simulink library "RollHeave_Decoupled"  (R2025a)
settings: Solver=VariableStepAuto  StartTime=0.0  StopTime=10.0  RelTol=1e-3
undefined symbols (not defined in the file): Linkage, Visual, X, Y, Z
libraries: Suspension_Utilities x12, sm_lib x8, nesl_utility x4, Linkage_Shock x2
Description:
  | Component of Simscape Vehicle Templates Library
  | 
  | Copyright 2018-2026 The MathWorks, Inc.
settings Model: Creator=smiller  LastModifiedBy=smiller
settings SolverCC: AlgebraicLoopSolver=TrustRegion
settings DataIOCC: ReturnWorkspaceOutputs=off
settings OptimizationCC: ReuseModelBlockBuffer=off
settings DebuggingCC: UnconnectedInputMsg=warning  UnconnectedOutputMsg=warning  UnconnectedLineMsg=warning  ArithmeticOperatorsInVariantConditions=warning
settings ModelReferenceCC: EnableRefExpFcnMdlSchedulingChecks=on
settings SFSimCC: CustomCodeUndefinedFunction=UseInterfaceOnly
settings RTWCC: GPUComputeCapability=3.5

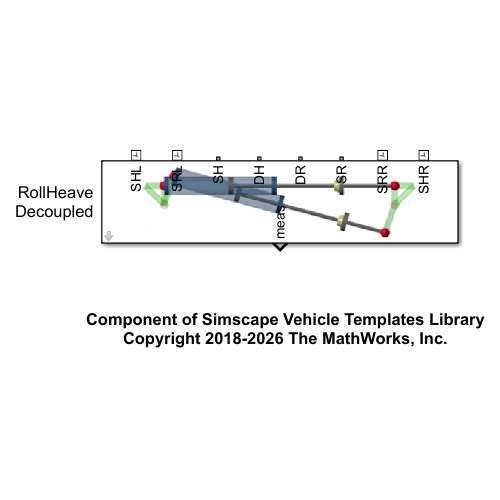
[thumbnail: Simulink's stored preview of the top-level diagram]
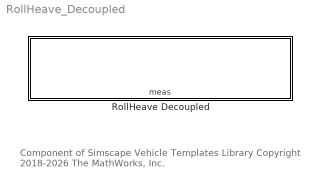
== system RollHeave_Decoupled ==
  note: Component of Simscape Vehicle Templates Library
      | Copyright 2018-2026 The MathWorks, Inc.
  RollHeave Decoupled : Subsystem  VariantControl=Variant1  mask(Roll and Heave Spring Dampers){hp_pushrod=Linkage.Pushrod.sBellcrank.Value, hp_bcr_pivot=Linkage.Bellcrank.sPivot.Value, hp_bcr_shock_heaveL=Linkage.Shock.Heave.sLeft.Value, hp_bcr_shock_heaveR=Linkage.Shock.Heave.sRight.Value, hp_bcr_shock_rollL=Linkage.Shock.Roll.sLeft.Value, hp_bcr_shock_rollR=Linkage.Shock.Roll.sRight.Value, shock_pist_mass_heave=Linkage.Shock.Heave.mPiston.Value, shock_pist_mass_roll=Linkage.Shock.Roll.mPiston.Value, shock_cyl_mass_heave=Linkage.Shock.Heave.mCylinder.Value, shock_cyl_mass_roll=Linkage.Shock.Roll.mCylinder.Value, up_lim_bumpstop_heave=Linkage.Endstop.Heave.xMax.Value, up_lim_bumpstop_roll=Linkage.Endstop.Roll.xMax.Value, low_lim_bumpstop_heave=Linkage.Endstop.Heave.xMin.Value, low_lim_bumpstop_roll=Linkage.Endstop.Roll.xMin.Value, clr_conn_shock=Visual.hp.clr, opc_conn_shock=Visual.hp.opc, size_conn_shock=Visual.hp.rad, clr_shock_cyl=Visual.Shock.cyl.clr, opc_shock_cyl=Visual.part.opc, radius_shock_cyl=Visual.Shock.cyl.rad, clr_shock_piston=Visual.Shock.piston.clr, opc_shock_piston=Visual.part.opc, clr_shock_bumpstop=Visual.Shock.bumpstop.clr, opc_shock_bumpstop=Visual.part.opc, deadvol_len_shock_cyl=Visual.Shock.dead_length, piston_len_shock=Visual.Shock.piston.len, cyl_cap_len_shock=Visual.Shock.cap.len, bumpstop_len_shock=Visual.Shock.bumpstop.len}
      mask prompts: hp_pushrod "HP Pushrod Inner  [xyz] (m)"; hp_bcr_pivot "HP Bellcrank Pivot [xyz] (m)"; deadvol_len_shock_cyl "Dead Volume Height (m)"; piston_len_shock "Piston Length (m)"; cyl_cap_len_shock "Cylinder Cap Length (m)"; bumpstop_len_shock "Bumpstop Length (m)"
      mask help: Models springs and dampers in a suspension design that decouples stiffness and damping for body roll and heave.
      mask init:
      | % Code to mirror hardpoint about vehicle xz plane
      | % and the plane defined by the bellcrank pivot axis
      | % and the y axis of the vehicle
      | % Code not used so that points can be specified independently
      | % Left here as a reference.
      | %{
      |  
      | a1 = atan2(hp_pushrod(1)-hp_bcr_pivot(1)   ,hp_pushrod(3)-hp_bcr_pivot(3));
      | a2 = atan2(hp_bcr_shock_roll(1)-hp_bcr_pivot(1),hp_bcr_shock_roll(3)-hp_bcr_pivot(3));
      | d_roll2piv = norm(hp_bcr_shock_roll([1 3])-hp_bcr_pivot([1 3]));
      | d_roll_mirror_axis = d_roll2piv*cos(a2-a1);
      | mirr_dx = d_roll_mirror_axis*sin(a1);
      | mirr_dz = d_roll_mirror_axis*cos(a1);
      | hp_bcr_shock_roll_r = ...
      |     [hp_bcr_shock_roll(1)-2*mirr_dx -hp_bcr_shock_roll(2) hp_bcr_shock_roll(3)-2*mirr_dz]
      | %}
      mask TypeOptions shock_pist_mass_heave: Shock Heave/shock_pist_mass
      mask TypeOptions shock_pist_mass_roll: Shock Roll/shock_pist_mass
      mask TypeOptions shock_cyl_mass_heave: Shock Heave/shock_cyl_mass
      mask TypeOptions shock_cyl_mass_roll: Shock Roll/shock_cyl_mass
      mask TypeOptions up_lim_bumpstop_heave: Shock Heave/up_lim_bumpstop
      mask TypeOptions up_lim_bumpstop_roll: Shock Roll/up_lim_bumpstop
      mask TypeOptions low_lim_bumpstop_heave: Shock Heave/low_lim_bumpstop
      mask TypeOptions low_lim_bumpstop_roll: Shock Roll/low_lim_bumpstop
      mask TypeOptions clr_conn_shock: Shock Heave/clr_conn_shock | Shock Roll/clr_conn_shock
      mask TypeOptions opc_conn_shock: Shock Heave/opc_conn_shock | Shock Roll/opc_conn_shock
      mask TypeOptions size_conn_shock: Shock Heave/size_conn_shock | Shock Roll/size_conn_shock
      mask TypeOptions clr_shock_cyl: Shock Heave/clr_shock_cyl | Shock Roll/clr_shock_cyl
      mask TypeOptions opc_shock_cyl: Shock Heave/opc_shock_cyl | Shock Roll/opc_shock_cyl
      mask TypeOptions radius_shock_cyl: Shock Heave/radius_shock_cyl | Shock Roll/radius_shock_cyl
      mask TypeOptions clr_shock_piston: Shock Heave/clr_shock_piston | Shock Roll/clr_shock_piston
      mask TypeOptions opc_shock_piston: Shock Heave/opc_shock_piston | Shock Roll/opc_shock_piston
      mask TypeOptions clr_shock_bumpstop: Shock Heave/clr_shock_bumpstop | Shock Roll/clr_shock_bumpstop
      mask TypeOptions opc_shock_bumpstop: Shock Heave/opc_shock_bumpstop | Shock Roll/opc_shock_bumpstop
      mask TypeOptions deadvol_len_shock_cyl: Shock Heave/deadvol_len_shock_cyl | Shock Roll/deadvol_len_shock_cyl
      mask TypeOptions piston_len_shock: Shock Heave/piston_len_shock | Shock Roll/piston_len_shock
      mask TypeOptions cyl_cap_len_shock: Shock Heave/cyl_cap_len_shock | Shock Roll/cyl_cap_len_shock
      mask TypeOptions bumpstop_len_shock: Shock Heave/bumpstop_len_shock | Shock Roll/bumpstop_len_shock
      mask DialogControl cont_hp Prompt: Hardpoints
      mask DialogControl text_hp_left Prompt: Left
      mask DialogControl text_hp_right Prompt: Right
      mask DialogControl text_hp_heave Prompt: Heave [xyz] (m)
      mask DialogControl text_hp_roll Prompt: Roll [xyz] (m)
      mask DialogControl cont_shock Prompt: Shock
      mask DialogControl text_shock_parts_blank Prompt: Parts
      mask DialogControl text_shock_heave Prompt: Heave
      mask DialogControl text_shock_roll Prompt: Roll
      mask DialogControl text_shock_pistm Prompt: Piston Mass (kg)
      mask DialogControl text_shock_cylm Prompt: Cylinder Mass (kg)
      mask DialogControl text_shock_bumpstop_par Prompt: Bumpstop
      mask DialogControl text_bump_ul Prompt: Upper Limit (m)
      mask DialogControl text_bump_low Prompt: Lower Limit (m)
      mask DialogControl cont_vis_shock Prompt: Visualization
      mask DialogControl text_clr_shock Prompt: Color  [RGB]
      mask DialogControl text_opc_shock Prompt: Opac. (0-1)
      mask DialogControl text_size_shock Prompt: Size (m)
      mask DialogControl text_conn_shock Prompt: Connections
      mask DialogControl text_shock_shock Prompt: Cylinder
      mask DialogControl text_shock_piston Prompt: Piston
      mask DialogControl text_piston_radius Prompt: <cylinder radius>
      mask DialogControl text_shock_bumpstop Prompt: Bumpstop
      mask DialogControl text_bumpstop_radius Prompt: <cylinder radius>
      mask Display: image('sm_car_vehicle_linkage_rollHeaveDecouple_IMAGE.png');

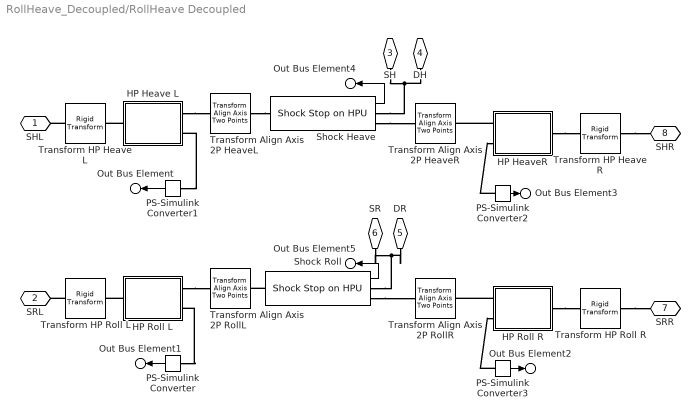
== system RollHeave_Decoupled/RollHeave Decoupled ==
  HP Heave L : Subsystem  mask(Revolute Joint 3 Points){popup_leftRight=Left, hp_bcr_pivot=hp_bcr_pivot, hp_pushrod_in=hp_pushrod, hp_bcr_shock=hp_bcr_shock_heaveL}
      mask prompts: popup_leftRight "Left/Right"; hp_bcr_pivot "HP Bellcrank Pivot [xyz] (m)"; hp_pushrod_in "HP Pushrod Inner [xyz] (m)"; hp_bcr_shock "HP Bellcrank Shock Heave [xyz] (m)"
      mask help: Revolute Joint with degree of freedom normal to 3 hardpoints.
      mask init:
      | % Set parameter for mirroring (+y or -y)
      | if(popup_leftRight == 1)
      |     rhs_susp = 1;    
      | elseif(popup_leftRight == 2)
      |     rhs_susp = -1;
      | end
      | 
      | rhs_hp = [1 rhs_susp 1];
      mask TypeOptions popup_leftRight: Left | Right
      mask Display: image('sm_car_variant_revolute.png')
  HP HeaveR : Subsystem  mask(Revolute Joint 3 Points){popup_leftRight=Right, hp_bcr_pivot=hp_bcr_pivot, hp_pushrod_in=hp_pushrod, hp_bcr_shock=hp_bcr_shock_heaveR}
      mask prompts: popup_leftRight "Left/Right"; hp_bcr_pivot "HP Bellcrank Pivot [xyz] (m)"; hp_pushrod_in "HP Pushrod Inner [xyz] (m)"; hp_bcr_shock "HP Bellcrank Shock Heave [xyz] (m)"
      mask help: Revolute Joint with degree of freedom normal to 3 hardpoints.
      mask init:
      | % Set parameter for mirroring (+y or -y)
      | if(popup_leftRight == 1)
      |     rhs_susp = 1;    
      | elseif(popup_leftRight == 2)
      |     rhs_susp = -1;
      | end
      | 
      | rhs_hp = [1 rhs_susp 1];
      mask TypeOptions popup_leftRight: Left | Right
      mask Display: image('sm_car_variant_revolute.png')
  HP Roll L : Subsystem  mask(Revolute Joint 3 Points){popup_leftRight=Left, hp_bcr_pivot=hp_bcr_pivot, hp_pushrod_in=hp_pushrod, hp_bcr_shock=hp_bcr_shock_heaveL}
      mask prompts: popup_leftRight "Left/Right"; hp_bcr_pivot "HP Bellcrank Pivot [xyz] (m)"; hp_pushrod_in "HP Pushrod Inner [xyz] (m)"; hp_bcr_shock "HP Bellcrank Shock Heave [xyz] (m)"
      mask help: Revolute Joint with degree of freedom normal to 3 hardpoints.
      mask init:
      | % Set parameter for mirroring (+y or -y)
      | if(popup_leftRight == 1)
      |     rhs_susp = 1;    
      | elseif(popup_leftRight == 2)
      |     rhs_susp = -1;
      | end
      | 
      | rhs_hp = [1 rhs_susp 1];
      mask TypeOptions popup_leftRight: Left | Right
      mask Display: image('sm_car_variant_revolute.png')
  HP Roll R : Subsystem  mask(Revolute Joint 3 Points){popup_leftRight=Right, hp_bcr_pivot=hp_bcr_pivot, hp_pushrod_in=hp_pushrod, hp_bcr_shock=hp_bcr_shock_heaveR}
      mask prompts: popup_leftRight "Left/Right"; hp_bcr_pivot "HP Bellcrank Pivot [xyz] (m)"; hp_pushrod_in "HP Pushrod Inner [xyz] (m)"; hp_bcr_shock "HP Bellcrank Shock Heave [xyz] (m)"
      mask help: Revolute Joint with degree of freedom normal to 3 hardpoints.
      mask init:
      | % Set parameter for mirroring (+y or -y)
      | if(popup_leftRight == 1)
      |     rhs_susp = 1;    
      | elseif(popup_leftRight == 2)
      |     rhs_susp = -1;
      | end
      | 
      | rhs_hp = [1 rhs_susp 1];
      mask TypeOptions popup_leftRight: Left | Right
      mask Display: image('sm_car_variant_revolute.png')
  PS-Simulink Converter{,1..3} (4 alike) : nesl_utility/PS-Simulink Converter  PhysicalDomain=network_engine_domain  SubClassName=ps_output  LeftPortType=input  RightPortType=output  PseudoPeriodic=off  Frequencies=[]  VectorFormat=1-D array  Unit=1  AffineConversion=off
  Shock Heave : Linkage_Shock/Shock Stop on HPU  shock_pist_mass=shock_pist_mass_heave  shock_cyl_mass=shock_cyl_mass_heave  hp_spr_top=hp_bcr_shock_heaveR  hp_spr_bot=hp_bcr_shock_heaveL  up_lim_bumpstop=up_lim_bumpstop_heave  low_lim_bumpstop=low_lim_bumpstop_heave  clr_conn_shock=clr_conn_shock  opc_conn_shock=opc_conn_shock  size_conn_shock=size_conn_shock  clr_shock_cyl=clr_shock_cyl  opc_shock_cyl=opc_shock_cyl  radius_shock_cyl=radius_shock_cyl  clr_shock_piston=clr_shock_piston  opc_shock_piston=opc_shock_piston  clr_shock_bumpstop=clr_shock_bumpstop  opc_shock_bumpstop=opc_shock_bumpstop  deadvol_len_shock_cyl=deadvol_len_shock_cyl  piston_len_shock=piston_len_shock  cyl_cap_len_shock=cyl_cap_len_shock  bumpstop_len_shock=bumpstop_len_shock
  Shock Roll : Linkage_Shock/Shock Stop on HPU  shock_pist_mass=shock_pist_mass_roll  shock_cyl_mass=shock_cyl_mass_roll  hp_spr_top=hp_bcr_shock_rollR  hp_spr_bot=hp_bcr_shock_rollL  up_lim_bumpstop=up_lim_bumpstop_roll  low_lim_bumpstop=low_lim_bumpstop_roll  clr_conn_shock=clr_conn_shock  opc_conn_shock=opc_conn_shock  size_conn_shock=size_conn_shock  clr_shock_cyl=clr_shock_cyl  opc_shock_cyl=opc_shock_cyl  radius_shock_cyl=radius_shock_cyl  clr_shock_piston=clr_shock_piston  opc_shock_piston=opc_shock_piston  clr_shock_bumpstop=clr_shock_bumpstop  opc_shock_bumpstop=opc_shock_bumpstop  deadvol_len_shock_cyl=deadvol_len_shock_cyl  piston_len_shock=piston_len_shock  cyl_cap_len_shock=cyl_cap_len_shock  bumpstop_len_shock=bumpstop_len_shock
  Transform Align Axis 2P HeaveL : Suspension_Utilities/Transform Align Axis Two Points  hp_b=hp_bcr_shock_heaveL  hp_t=hp_bcr_shock_heaveR  popup_f_axis=+Z
  Transform Align Axis 2P HeaveR : Suspension_Utilities/Transform Align Axis Two Points  hp_b=hp_bcr_shock_heaveR  hp_t=hp_bcr_shock_heaveL  popup_f_axis=-Z
  Transform Align Axis 2P RollL : Suspension_Utilities/Transform Align Axis Two Points  hp_b=hp_bcr_shock_rollL  hp_t=hp_bcr_shock_rollR  popup_f_axis=+Z
  Transform Align Axis 2P RollR : Suspension_Utilities/Transform Align Axis Two Points  hp_b=hp_bcr_shock_rollR  hp_t=hp_bcr_shock_rollL  popup_f_axis=-Z
  "Transform HP Heave L " : sm_lib/Frames and Transforms/Rigid Transform  RotationMethod=None  FollAlignAxisA=+X  BaseAlignAxisA=+Y  FollAlignAxisB=+Y  BaseAlignAxisB=+Z  RotationStandardAxis=+Z  RotationAngle=0.0  RotationAngleUnits=deg  RotationArbitraryAxis=[0 0 1]  RotationSequenceAxes=FollowerAxes  RotationSequence=XYX  RotationSequenceAngles=[0 0 0]  RotationSequenceAnglesUnits=deg  RotationMatrix=[1 0 0; 0 1 0; 0 0 1]  Quaternion=[1 0 0 0]  TranslationMethod=Cartesian  TranslationCartesianOffset=hp_bcr_shock_heaveL  TranslationCartesianOffsetUnits=m  TranslationStandardAxis=+Z  TranslationStandardOffset=0  TranslationStandardOffsetUnits=m  TranslationROffset=0  TranslationROffsetUnits=m  TranslationThetaOffset=0  TranslationThetaOffsetUnits=deg  TranslationZOffset=0  TranslationZOffsetUnits=m
  Transform HP Heave R : sm_lib/Frames and Transforms/Rigid Transform  RotationMethod=None  FollAlignAxisA=+X  BaseAlignAxisA=+Y  FollAlignAxisB=+Y  BaseAlignAxisB=+Z  RotationStandardAxis=+Z  RotationAngle=0.0  RotationAngleUnits=deg  RotationArbitraryAxis=[0 0 1]  RotationSequenceAxes=FollowerAxes  RotationSequence=XYX  RotationSequenceAngles=[0 0 0]  RotationSequenceAnglesUnits=deg  RotationMatrix=[1 0 0; 0 1 0; 0 0 1]  Quaternion=[1 0 0 0]  TranslationMethod=Cartesian  TranslationCartesianOffset=hp_bcr_shock_heaveR  TranslationCartesianOffsetUnits=m  TranslationStandardAxis=+Z  TranslationStandardOffset=0  TranslationStandardOffsetUnits=m  TranslationROffset=0  TranslationROffsetUnits=m  TranslationThetaOffset=0  TranslationThetaOffsetUnits=deg  TranslationZOffset=0  TranslationZOffsetUnits=m
  Transform HP Roll L : sm_lib/Frames and Transforms/Rigid Transform  RotationMethod=None  FollAlignAxisA=+X  BaseAlignAxisA=+Y  FollAlignAxisB=+Y  BaseAlignAxisB=+Z  RotationStandardAxis=+Z  RotationAngle=0.0  RotationAngleUnits=deg  RotationArbitraryAxis=[0 0 1]  RotationSequenceAxes=FollowerAxes  RotationSequence=XYX  RotationSequenceAngles=[0 0 0]  RotationSequenceAnglesUnits=deg  RotationMatrix=[1 0 0; 0 1 0; 0 0 1]  Quaternion=[1 0 0 0]  TranslationMethod=Cartesian  TranslationCartesianOffset=hp_bcr_shock_rollL  TranslationCartesianOffsetUnits=m  TranslationStandardAxis=+Z  TranslationStandardOffset=0  TranslationStandardOffsetUnits=m  TranslationROffset=0  TranslationROffsetUnits=m  TranslationThetaOffset=0  TranslationThetaOffsetUnits=deg  TranslationZOffset=0  TranslationZOffsetUnits=m
  Transform HP Roll R : sm_lib/Frames and Transforms/Rigid Transform  RotationMethod=None  FollAlignAxisA=+X  BaseAlignAxisA=+Y  FollAlignAxisB=+Y  BaseAlignAxisB=+Z  RotationStandardAxis=+Z  RotationAngle=0.0  RotationAngleUnits=deg  RotationArbitraryAxis=[0 0 1]  RotationSequenceAxes=FollowerAxes  RotationSequence=XYX  RotationSequenceAngles=[0 0 0]  RotationSequenceAnglesUnits=deg  RotationMatrix=[1 0 0; 0 1 0; 0 0 1]  Quaternion=[1 0 0 0]  TranslationMethod=Cartesian  TranslationCartesianOffset=hp_bcr_shock_rollR  TranslationCartesianOffsetUnits=m  TranslationStandardAxis=+Z  TranslationStandardOffset=0  TranslationStandardOffsetUnits=m  TranslationROffset=0  TranslationROffsetUnits=m  TranslationThetaOffset=0  TranslationThetaOffsetUnits=deg  TranslationZOffset=0  TranslationZOffsetUnits=m
  SHL : PMIOPort  Side=Left
  SRL : PMIOPort  Port=2  Side=Left
  SH : PMIOPort  Port=3  Side=Left
  DH : PMIOPort  Port=4  Side=Left
  DR : PMIOPort  Port=5  Side=Left
  SR : PMIOPort  Port=6  Side=Left
  SRR : PMIOPort  Port=7  Side=Left
  SHR : PMIOPort  Port=8  Side=Left
  Out Bus Element : Outport  VectorParamsAs1DForOutWhenUnconnected=off  PortName=meas  Element=qHL
  Out Bus Element3 : Outport  VectorParamsAs1DForOutWhenUnconnected=off  PortName=meas  Element=qHR
  Out Bus Element1 : Outport  VectorParamsAs1DForOutWhenUnconnected=off  PortName=meas  Element=qRL
  Out Bus Element2 : Outport  VectorParamsAs1DForOutWhenUnconnected=off  PortName=meas  Element=qRR
  Out Bus Element4 : Outport  VectorParamsAs1DForOutWhenUnconnected=off  PortName=meas  Element=xHeave
  Out Bus Element5 : Outport  VectorParamsAs1DForOutWhenUnconnected=off  PortName=meas  Element=xRoll
  wires:
  PS-Simulink Converter/1 -> Out Bus Element1/1
  PS-Simulink Converter1/1 -> Out Bus Element/1
  PS-Simulink Converter2/1 -> Out Bus Element3/1
  PS-Simulink Converter3/1 -> Out Bus Element2/1
  Shock Heave/1 -> Out Bus Element4/1
  Shock Roll/1 -> Out Bus Element5/1
  connections:
  "Transform HP Heave L "/LConn1 -- SHL/RConn1
  Transform Align Axis 2P HeaveL/RConn1 -- Shock Heave/LConn1
  Transform HP Heave R/LConn1 -- SHR/RConn1
  HP HeaveR/LConn1 -- Transform HP Heave R/RConn1
  HP HeaveR/RConn1 -- Transform Align Axis 2P HeaveR/LConn1
  HP Heave L/LConn1 -- "Transform HP Heave L "/RConn1
  SH/RConn1 -- Shock Heave/RConn1 -- DH/RConn1
  DR/RConn1 -- SR/RConn1 -- Shock Roll/RConn1
  HP Roll R/RConn1 -- Transform Align Axis 2P RollR/LConn1
  Transform HP Roll R/LConn1 -- SRR/RConn1
  HP Roll L/RConn1 -- Transform Align Axis 2P RollL/LConn1
  Transform HP Roll L/LConn1 -- SRL/RConn1
  HP Roll L/LConn1 -- Transform HP Roll L/RConn1
  HP Roll R/LConn1 -- Transform HP Roll R/RConn1
  Shock Roll/RConn2 -- Transform Align Axis 2P RollR/RConn1
  Shock Roll/LConn1 -- Transform Align Axis 2P RollL/RConn1
  Shock Heave/RConn2 -- Transform Align Axis 2P HeaveR/RConn1
  HP Heave L/RConn1 -- Transform Align Axis 2P HeaveL/LConn1
  PS-Simulink Converter/LConn1 -- HP Roll L/RConn2
  PS-Simulink Converter1/LConn1 -- HP Heave L/RConn2
  PS-Simulink Converter2/LConn1 -- HP HeaveR/RConn2
  PS-Simulink Converter3/LConn1 -- HP Roll R/RConn2

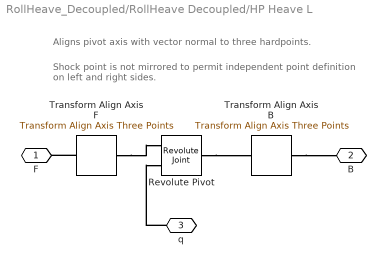
== system RollHeave_Decoupled/RollHeave Decoupled/HP Heave L ==
  note: Shock point is not mirrored to permit independent point definition on left and right sides.
  note: Aligns pivot axis with vector normal to three hardpoints.
  Revolute Pivot : sm_lib/Joints/Revolute Joint  JointMode=Normal  CompositeWrenchDir=FollowerOnBase  CompositeWrenchFrame=BaseFrame  SenseConstraintForce=off  SenseConstraintTorque=off  SenseTotalForce=off  SenseTotalTorque=off  PositionTargetSpecify=off  PositionTargetPriority=Low  PositionTargetValue=0  PositionTargetValueUnits=deg  VelocityTargetSpecify=off  VelocityTargetPriority=High  VelocityTargetValue=0  VelocityTargetValueUnits=deg/s  EquilibriumPosition=0  EquilibriumPositionUnits=deg  SpringStiffness=0  SpringStiffnessUnits=N*m/deg  DampingCoefficient=0  DampingCoefficientUnits=N*m/(deg/s)  LowerLimitSpecify=off  LowerLimitBound=-90  LowerLimitBoundUnits=deg  LowerLimitStiffness=1e4  LowerLimitStiffnessUnits=N*m/deg  LowerLimitDamping=10  LowerLimitDampingUnits=N*m/(deg/s)  LowerLimitTransitionRegionWidth=0.1  LowerLimitTransitionRegionWidthUnits=deg  UpperLimitSpecify=off  UpperLimitBound=90  UpperLimitBoundUnits=deg  UpperLimitStiffness=1e4  UpperLimitStiffnessUnits=N*m/deg  UpperLimitDamping=10  UpperLimitDampingUnits=N*m/(deg/s)  UpperLimitTransitionRegionWidth=0.1  UpperLimitTransitionRegionWidthUnits=deg  TorqueActuationMode=NoTorque  MotionActuationMode=ComputedMotion  SensePosition=on  SenseVelocity=off  SenseAcceleration=off  SenseTorqueForce=off  SenseLowerLimitTorqueForce=off  SenseUpperLimitTorqueForce=off
  Transform Align Axis B : Suspension_Utilities/Transform Align Axis Three Points  pt1=hp_bcr_pivot.*rhs_hp  pt2=hp_pushrod_in.*rhs_hp  pt3=hp_bcr_shock  popup_f_axis=+Z
  Transform Align Axis F : Suspension_Utilities/Transform Align Axis Three Points  pt1=hp_bcr_pivot.*rhs_hp  pt2=hp_pushrod_in.*rhs_hp  pt3=hp_bcr_shock  popup_f_axis=+Z
  F : PMIOPort  Side=Right
  B : PMIOPort  Port=2  Side=Left
  q : PMIOPort  Port=3  Side=Right
  connections:
  Transform Align Axis B/LConn1 -- B/RConn1
  Transform Align Axis F/RConn1 -- Revolute Pivot/RConn1
  Revolute Pivot/LConn1 -- Transform Align Axis B/RConn1
  Transform Align Axis F/LConn1 -- F/RConn1
  q/RConn1 -- Revolute Pivot/RConn2

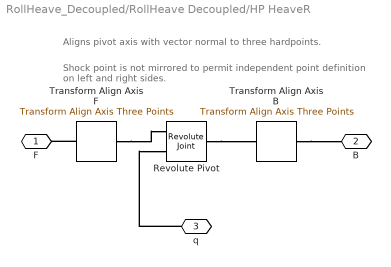
== system RollHeave_Decoupled/RollHeave Decoupled/HP HeaveR ==
  note: Shock point is not mirrored to permit independent point definition on left and right sides.
  note: Aligns pivot axis with vector normal to three hardpoints.
  Revolute Pivot : sm_lib/Joints/Revolute Joint  JointMode=Normal  CompositeWrenchDir=FollowerOnBase  CompositeWrenchFrame=BaseFrame  SenseConstraintForce=off  SenseConstraintTorque=off  SenseTotalForce=off  SenseTotalTorque=off  PositionTargetSpecify=off  PositionTargetPriority=Low  PositionTargetValue=0  PositionTargetValueUnits=deg  VelocityTargetSpecify=off  VelocityTargetPriority=High  VelocityTargetValue=0  VelocityTargetValueUnits=deg/s  EquilibriumPosition=0  EquilibriumPositionUnits=deg  SpringStiffness=0  SpringStiffnessUnits=N*m/deg  DampingCoefficient=0  DampingCoefficientUnits=N*m/(deg/s)  LowerLimitSpecify=off  LowerLimitBound=-90  LowerLimitBoundUnits=deg  LowerLimitStiffness=1e4  LowerLimitStiffnessUnits=N*m/deg  LowerLimitDamping=10  LowerLimitDampingUnits=N*m/(deg/s)  LowerLimitTransitionRegionWidth=0.1  LowerLimitTransitionRegionWidthUnits=deg  UpperLimitSpecify=off  UpperLimitBound=90  UpperLimitBoundUnits=deg  UpperLimitStiffness=1e4  UpperLimitStiffnessUnits=N*m/deg  UpperLimitDamping=10  UpperLimitDampingUnits=N*m/(deg/s)  UpperLimitTransitionRegionWidth=0.1  UpperLimitTransitionRegionWidthUnits=deg  TorqueActuationMode=NoTorque  MotionActuationMode=ComputedMotion  SensePosition=on  SenseVelocity=off  SenseAcceleration=off  SenseTorqueForce=off  SenseLowerLimitTorqueForce=off  SenseUpperLimitTorqueForce=off
  Transform Align Axis B : Suspension_Utilities/Transform Align Axis Three Points  pt1=hp_bcr_pivot.*rhs_hp  pt2=hp_pushrod_in.*rhs_hp  pt3=hp_bcr_shock  popup_f_axis=+Z
  Transform Align Axis F : Suspension_Utilities/Transform Align Axis Three Points  pt1=hp_bcr_pivot.*rhs_hp  pt2=hp_pushrod_in.*rhs_hp  pt3=hp_bcr_shock  popup_f_axis=+Z
  F : PMIOPort  Side=Right
  B : PMIOPort  Port=2  Side=Left
  q : PMIOPort  Port=3  Side=Right
  connections:
  Transform Align Axis F/LConn1 -- F/RConn1
  Revolute Pivot/LConn1 -- Transform Align Axis B/RConn1
  Transform Align Axis F/RConn1 -- Revolute Pivot/RConn1
  Transform Align Axis B/LConn1 -- B/RConn1
  q/RConn1 -- Revolute Pivot/RConn2

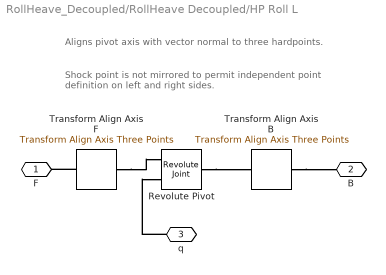
== system RollHeave_Decoupled/RollHeave Decoupled/HP Roll L ==
  note: Shock point is not mirrored to permit independent point definition on left and right sides.
  note: Aligns pivot axis with vector normal to three hardpoints.
  Revolute Pivot : sm_lib/Joints/Revolute Joint  JointMode=Normal  CompositeWrenchDir=FollowerOnBase  CompositeWrenchFrame=BaseFrame  SenseConstraintForce=off  SenseConstraintTorque=off  SenseTotalForce=off  SenseTotalTorque=off  PositionTargetSpecify=off  PositionTargetPriority=Low  PositionTargetValue=0  PositionTargetValueUnits=deg  VelocityTargetSpecify=off  VelocityTargetPriority=High  VelocityTargetValue=0  VelocityTargetValueUnits=deg/s  EquilibriumPosition=0  EquilibriumPositionUnits=deg  SpringStiffness=0  SpringStiffnessUnits=N*m/deg  DampingCoefficient=0  DampingCoefficientUnits=N*m/(deg/s)  LowerLimitSpecify=off  LowerLimitBound=-90  LowerLimitBoundUnits=deg  LowerLimitStiffness=1e4  LowerLimitStiffnessUnits=N*m/deg  LowerLimitDamping=10  LowerLimitDampingUnits=N*m/(deg/s)  LowerLimitTransitionRegionWidth=0.1  LowerLimitTransitionRegionWidthUnits=deg  UpperLimitSpecify=off  UpperLimitBound=90  UpperLimitBoundUnits=deg  UpperLimitStiffness=1e4  UpperLimitStiffnessUnits=N*m/deg  UpperLimitDamping=10  UpperLimitDampingUnits=N*m/(deg/s)  UpperLimitTransitionRegionWidth=0.1  UpperLimitTransitionRegionWidthUnits=deg  TorqueActuationMode=NoTorque  MotionActuationMode=ComputedMotion  SensePosition=on  SenseVelocity=off  SenseAcceleration=off  SenseTorqueForce=off  SenseLowerLimitTorqueForce=off  SenseUpperLimitTorqueForce=off
  Transform Align Axis B : Suspension_Utilities/Transform Align Axis Three Points  pt1=hp_bcr_pivot.*rhs_hp  pt2=hp_pushrod_in.*rhs_hp  pt3=hp_bcr_shock  popup_f_axis=+Z
  Transform Align Axis F : Suspension_Utilities/Transform Align Axis Three Points  pt1=hp_bcr_pivot.*rhs_hp  pt2=hp_pushrod_in.*rhs_hp  pt3=hp_bcr_shock  popup_f_axis=+Z
  F : PMIOPort  Side=Right
  B : PMIOPort  Port=2  Side=Left
  q : PMIOPort  Port=3  Side=Right
  connections:
  Transform Align Axis F/LConn1 -- F/RConn1
  Revolute Pivot/LConn1 -- Transform Align Axis B/RConn1
  Transform Align Axis F/RConn1 -- Revolute Pivot/RConn1
  Transform Align Axis B/LConn1 -- B/RConn1
  q/RConn1 -- Revolute Pivot/RConn2

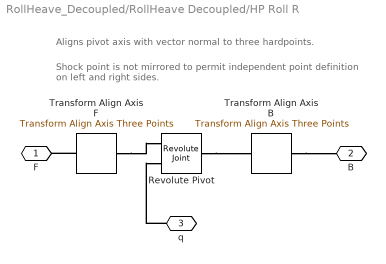
== system RollHeave_Decoupled/RollHeave Decoupled/HP Roll R ==
  note: Shock point is not mirrored to permit independent point definition on left and right sides.
  note: Aligns pivot axis with vector normal to three hardpoints.
  Revolute Pivot : sm_lib/Joints/Revolute Joint  JointMode=Normal  CompositeWrenchDir=FollowerOnBase  CompositeWrenchFrame=BaseFrame  SenseConstraintForce=off  SenseConstraintTorque=off  SenseTotalForce=off  SenseTotalTorque=off  PositionTargetSpecify=off  PositionTargetPriority=Low  PositionTargetValue=0  PositionTargetValueUnits=deg  VelocityTargetSpecify=off  VelocityTargetPriority=High  VelocityTargetValue=0  VelocityTargetValueUnits=deg/s  EquilibriumPosition=0  EquilibriumPositionUnits=deg  SpringStiffness=0  SpringStiffnessUnits=N*m/deg  DampingCoefficient=0  DampingCoefficientUnits=N*m/(deg/s)  LowerLimitSpecify=off  LowerLimitBound=-90  LowerLimitBoundUnits=deg  LowerLimitStiffness=1e4  LowerLimitStiffnessUnits=N*m/deg  LowerLimitDamping=10  LowerLimitDampingUnits=N*m/(deg/s)  LowerLimitTransitionRegionWidth=0.1  LowerLimitTransitionRegionWidthUnits=deg  UpperLimitSpecify=off  UpperLimitBound=90  UpperLimitBoundUnits=deg  UpperLimitStiffness=1e4  UpperLimitStiffnessUnits=N*m/deg  UpperLimitDamping=10  UpperLimitDampingUnits=N*m/(deg/s)  UpperLimitTransitionRegionWidth=0.1  UpperLimitTransitionRegionWidthUnits=deg  TorqueActuationMode=NoTorque  MotionActuationMode=ComputedMotion  SensePosition=on  SenseVelocity=off  SenseAcceleration=off  SenseTorqueForce=off  SenseLowerLimitTorqueForce=off  SenseUpperLimitTorqueForce=off
  Transform Align Axis B : Suspension_Utilities/Transform Align Axis Three Points  pt1=hp_bcr_pivot.*rhs_hp  pt2=hp_pushrod_in.*rhs_hp  pt3=hp_bcr_shock  popup_f_axis=+Z
  Transform Align Axis F : Suspension_Utilities/Transform Align Axis Three Points  pt1=hp_bcr_pivot.*rhs_hp  pt2=hp_pushrod_in.*rhs_hp  pt3=hp_bcr_shock  popup_f_axis=+Z
  F : PMIOPort  Side=Right
  B : PMIOPort  Port=2  Side=Left
  q : PMIOPort  Port=3  Side=Right
  connections:
  Transform Align Axis B/LConn1 -- B/RConn1
  Transform Align Axis F/RConn1 -- Revolute Pivot/RConn1
  Revolute Pivot/LConn1 -- Transform Align Axis B/RConn1
  Transform Align Axis F/LConn1 -- F/RConn1
  q/RConn1 -- Revolute Pivot/RConn2
